simulink model "quartercar_RL_6_no_G"  (R2023a)
settings: Solver=VariableStepAuto  StartTime=0  StopTime=10  FixedStep=0.05  RelTol=1e-5  EnableMultiTasking=on
model workspace (MAT data in the model file):
  cs = 2126
  ks = 24000
  kt = 243000
  ms = 365
  mu = 43
undefined symbols (not defined in the file or in its folder): magnitude
libraries: simulink x3, slpidlib x1, rllib x1
settings Model: Creator=Administrator  LastModifiedBy=Yuk
settings SolverCC: AllowMultiTaskInputOutput=on  InsertRTBMode=Never (minimum delay)
settings DataIOCC: SaveFormat=Array
settings OptimizationCC: LifeSpan=inf
settings DebuggingCC: AlgebraicLoopMsg=none  UnderspecifiedInitializationDetection=Classic  MergeDetectMultiDrivingBlocksExec=none  SolverPrmCheckMsg=warning  UnconnectedInputMsg=warning  UnconnectedOutputMsg=warning  UnconnectedLineMsg=warning  StateNameClashWarn=warning  SFUnexpectedBacktrackingDiag=warning  SFNoUnconditionalDefaultTransitionDiag=warning  SFExecutionAtInitializationDiag=none  ArithmeticOperatorsInVariantConditions=warning
settings HardwareCC: ProdBitPerPointer=32  ProdBitPerSizeT=32  ProdBitPerPtrDiffT=32  ProdLargestAtomicFloat=None  ProdIntDivRoundTo=Undefined  ProdEndianess=Unspecified  ProdWordSize=32  ProdHWDeviceType=32-bit Generic
settings ModelReferenceCC: PropagateSignalLabelsOutOfModel=off
settings SFSimCC: SimUseLocalCustomCode=off  CustomCodeUndefinedFunction=UseInterfaceOnly  SimTargetLang=C++
settings RTWCC: RTWUseLocalCustomCode=off
settings CodeAppCC: StateflowObjectComments=on
settings GRTTargetCC: TargetLangStandard=C89/C90 (ANSI)
settings ConfigComp: CovMetricSettings=dw  CovSaveCumulativeToWorkspaceVar=on  CovSaveSingleToWorkspaceVar=on  CovExternalEMLEnable=off

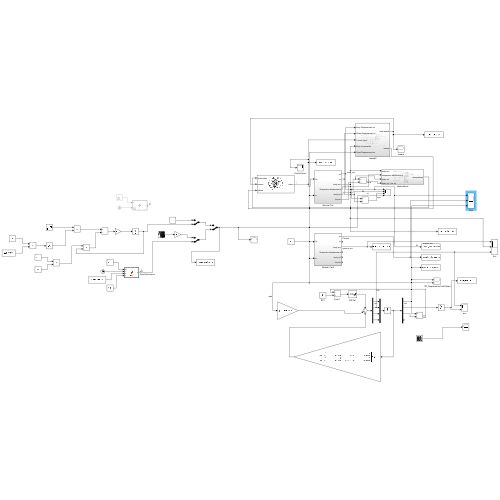
[thumbnail: Simulink's stored preview of the top-level diagram]
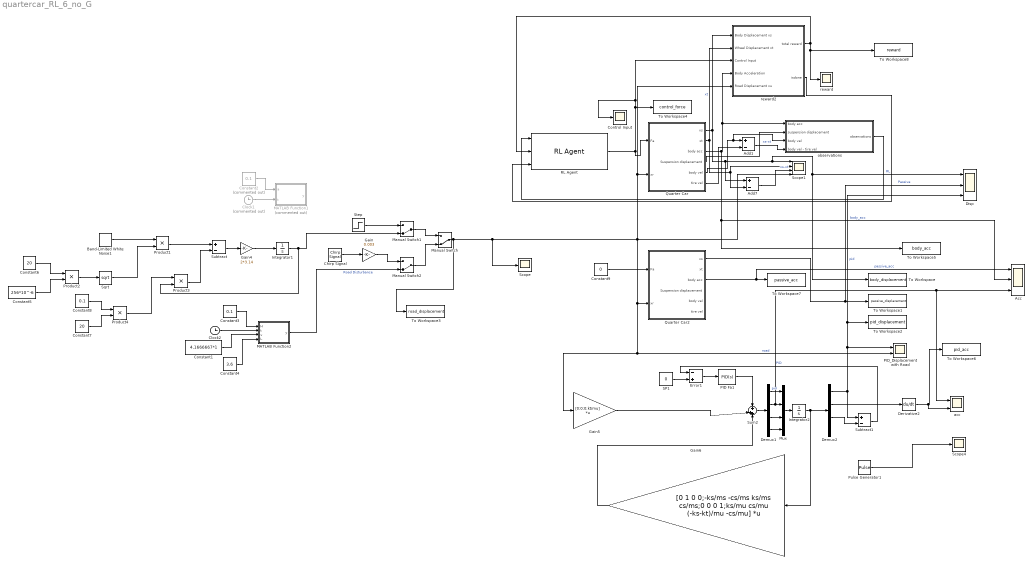
== system quartercar_RL_6_no_G ==
  Acc : Scope  NumInputPorts=3
  Add1 : Sum  Inputs=+-
  Add7 : Sum  Inputs=+-
  Band-Limited White Noise1 : simulink/Sources/Band-Limited White Noise  Cov=[5.4*10^-3]  Ts=0.1  seed=[23341]
  Chirp Signal : simulink/Sources/Chirp Signal  f1=1  T=10  f2=1
  Clock1 : Clock  Commented=on
  Clock2 : Clock
  Constant1 : Constant  Value=4.1666667*1
  Constant2 : Constant  Commented=on  Value=0.1
  Constant3 : Constant  Value=0.1
  Constant4 : Constant  Value=3.6
  Constant5 : Constant  Value=256*10^-6
  Constant6 : Constant  Value=20
  Constant7 : Constant  Value=20
  Constant8 : Constant  Value=0.1
  Constant9 : Constant  Value=0
  Control Input : Scope
  Demux1 : Demux
  Demux2 : Demux
  Derivative2 : Derivative
  Disp : Scope  NumInputPorts=3
  Error1 : Sum  Inputs=-+
  Gain : Gain  Gain=0.003
  Gain4 : Gain  Gain=2*3.14
  Gain5 : Gain  Gain=[0;0;0;kt/mu]  Multiplication=Matrix(K*u)
  Gain6 : Gain  Gain=[0 1 0 0;-ks/ms -cs/ms ks/ms cs/ms;0 0 0 1;ks/mu cs/mu (-ks-kt)/mu -cs/mu]  Multiplication=Matrix(K*u)
  Integrator1 : Integrator
  Integrator2 : Integrator
  MATLAB Function1 : MATLAB Function  Commented=on  TreatAsAtomicUnit=on
  MATLAB Function2 : MATLAB Function  TreatAsAtomicUnit=on
  Manual Switch : ManualSwitch  CurrentSetting=0
  Manual Switch1 : ManualSwitch  CurrentSetting=0
  Manual Switch2 : ManualSwitch  CurrentSetting=0
  Mux : Mux
  PID Fa1 : slpidlib/PID Controller  Controller=PID  Form=Parallel  TimeDomain=Continuous-time  UseExternalTs=off  SampleTime=1  IntegratorMethod=Forward Euler  FilterMethod=Forward Euler  ControllerParametersSource=internal  P=0.8  I=0.1  UseKiTs=off  D=0.5  N=100  UseFilter=on  TunerSelectOption=Transfer Function Based (PID Tuner App)  InitialConditionSource=internal  InitialConditionForIntegrator=0  InitialConditionForFilter=0  DifferentiatorICPrevScaledInput=0  ExternalReset=none  TrackingMode=off  Kt=1  LimitOutput=on  SatLimitsSource=internal  UpperSaturationLimit=4000  LowerSaturationLimit=-4000  LinearizeAsGain=off  AntiWindupMode=none  Kb=1  LimitIntegrator=off  UpperIntegratorSaturationLimit=inf  LowerIntegratorSaturationLimit=-inf  POutMin=[]  POutMax=[]  IOutMin=[]  IOutMax=[]  DOutMin=[]  DOutMax=[]  NOutMin=[]  NOutMax=[]  SumOutMin=[]  SumOutMax=[]  SaturationOutMin=[]  SaturationOutMax=[]  PParamMin=[]  PParamMax=[]  IParamMin=[]  IParamMax=[]  DParamMin=[]  DParamMax=[]  NParamMin=[]  NParamMax=[]  KbParamMin=[]  KbParamMax=[]  KtParamMin=[]  KtParamMax=[]  KbOutMin=[]  KbOutMax=[]  KtOutMin=[]  KtOutMax=[]  IntegratorOutMin=[]  IntegratorOutMax=[]  FilterOutMin=[]  FilterOutMax=[]  SumI1OutMin=[]  SumI1OutMax=[]  SumI2OutMin=[]  SumI2OutMax=[]  SumI3OutMin=[]  SumI3OutMax=[]  SumI4OutMin=[]  SumI4OutMax=[]  SumDOutMin=[]  SumDOutMax=[]  DifferentiatorOutMin=[]  DifferentiatorOutMax=[]  FilterDiffOutCoefMin=[]  FilterDiffOutCoefMax=[]  ReciprocalOutMin=[]  ReciprocalOutMax=[]  SumDenOutMin=[]  SumDenOutMax=[]  SumNumOutMin=[]  SumNumOutMax=[]  DivideOutMin=[]  DivideOutMax=[]  UdiffTsProdOutMin=[]  UdiffTsProdOutMax=[]  NTsProdOutMin=[]  NTsProdOutMax=[]  UintegralTsProdOutMin=[]  UintegralTsProdOutMax=[]  UngainTsProdOutMin=[]  UngainTsProdOutMax=[]  ClampingZeroOutDataTypeStr=Inherit: Inherit via back propagation  ClampingZeroOutMin=[]  ClampingZeroOutMax=[]  FilterDenConstantOutDataTypeStr=Inherit: Inherit via back propagation  FilterDenConstantOutMin=[]  FilterDenConstantOutMax=[]  PCopyOutDataTypeStr=Inherit: Inherit via back propagation  PCopyOutMin=[]  PCopyOutMax=[]  NCopyOutDataTypeStr=Inherit: Inherit via back propagation  NCopyOutMin=[]  NCopyOutMax=[]  IntegratorContinuousStateAttributes=''  IntegratorStateMustResolveToSignalObject=off  IntegratorRTWStateStorageClass=Auto  FilterContinuousStateAttributes=''  FilterStateMustResolveToSignalObject=off  FilterRTWStateStorageClass=Auto  ParallelPVariant=InternalParameters  IdealPVariant=Disabled  IVariant=InternalParameters  DVariant=InternalParameters  IntegratorVariant=Continuous  SatVariant=Enabled  AWVariant=Passthrough  PCopyVariant=Disabled  TRVariant=Disabled  FdbkBlocksVariant=Forward  IdealPFdbkVariant=Disabled  SatFdbkVariant=Disabled  DerivativeFilterVariant=ContFilter  NVariant=InternalParameters  NCopyVariant=Disabled  FilterICVariant=InternalICsFilter  IntegratorICVariant=InternalICs  ExternalResetVariant=Disabled  TRSumVariant=Passthrough  SumFdbkVariant=Disabled  SumVariant=Sum_PID  TsampFilterVariant=InternalTs  TsampNgainVariant=Passthrough  TsampIntegralVariant=Disabled_SignalSpec  ExternalSaturationOutDataTypeStr=Inherit: Same as second input
  PID_Displacement with Road : Scope  NumInputPorts=2
  Product{1..4} (4 alike) : Product
  Pulse Generator1 : DiscretePulseGenerator  PulseType=Time based  Period=10  PulseWidth=5
  Quarter Car : Subsystem
  Quarter Car2 : Subsystem
  RL Agent : rllib/RL Agent  Agent=saved_agent  ExternalActionAsInput=off  ProvideLastAction=off  ProvideCumRwd=off  TreatAsDirectFeedthrough=on  UseStrictObservationDataTypes=off
  SP1 : Constant  Value=0
  Scope : Scope
  Scope1 : Scope  NumInputPorts=4
  Scope4 : Scope
  Sqrt : Sqrt
  Step : Step  SampleTime=0
  Subtract : Sum  Inputs=+-
  Subtract1 : Sum  Inputs=+-
  Sum2 : Sum  Inputs=+|++
  To Workspace : ToWorkspace  VariableName=body_displacement  SaveFormat=Timeseries  SampleTime=-1
  To Workspace1 : ToWorkspace  VariableName=passive_displacement  SaveFormat=Timeseries  SampleTime=-1
  To Workspace2 : ToWorkspace  VariableName=pid_displacement  SaveFormat=Timeseries  SampleTime=-1
  To Workspace3 : ToWorkspace  VariableName=road_displacement  SaveFormat=Timeseries  SampleTime=-1
  To Workspace4 : ToWorkspace  VariableName=control_force  SaveFormat=Timeseries  SampleTime=-1
  To Workspace5 : ToWorkspace  VariableName=body_acc  SaveFormat=Timeseries  SampleTime=-1
  To Workspace6 : ToWorkspace  VariableName=pid_acc  SaveFormat=Timeseries  SampleTime=0.05
  To Workspace7 : ToWorkspace  VariableName=passive_acc  SaveFormat=Timeseries  SampleTime=-1
  To Workspace8 : ToWorkspace  VariableName=reward  SaveFormat=Timeseries  SampleTime=-1
  acc : Scope  NumInputPorts=2
  observations : Subsystem
  reward : Scope
  reward2 : Subsystem
  wires:
  Quarter Car/1(xs) -> reward2/1(Body Displacement xs), Add7/1, To Workspace/1, Disp/1, Scope1/1  "RL"
  Quarter Car/2(xt) -> Add7/2, Scope1/2, reward2/2(Wheel Displacement xt)  "xt"
  Add7/1 -> Scope1/3  "xs-xt"
  Constant2/1 -> MATLAB Function1/1(a)
  Clock1/1 -> MATLAB Function1/2(t)
  reward2/1(total reward) -> reward/1, To Workspace8/1, RL Agent/2
  Quarter Car/3(body acc) -> To Workspace5/1, Acc/2, reward2/4(Body Acceleration), observations/1(body acc)  "body_acc"
  observations/1(observations) -> RL Agent/1
  reward2/2(isdone) -> RL Agent/3
  Quarter Car/4(Suspension displacement) -> observations/2(suspension displacement)
  Quarter Car/5(body vel) -> observations/3(body vel), Add1/1
  Quarter Car/6(tire vel) -> Add1/2
  Add1/1 -> observations/4(body vel - tire vel)  "xs-xt"
  RL Agent/1 -> Quarter Car/1(Fa), To Workspace4/1, Control Input/1, reward2/3(Control Input)
  Quarter Car2/1(xs) -> Disp/2, To Workspace1/1  "Passive"
  Quarter Car2/3(body acc) -> Acc/1, To Workspace7/1  "passive_acc"
  Manual Switch1/1 -> Manual Switch/1
  Integrator1/1 -> Product3/2, Manual Switch1/2
  Constant5/1 -> Product2/2
  Sqrt/1 -> Product1/2
  Constant6/1 -> Product2/1
  Product2/1 -> Sqrt/1
  Constant7/1 -> Product4/2
  Gain4/1 -> Integrator1/1
  Product1/1 -> Subtract/1
  Band-Limited White Noise1/1 -> Product1/1
  Product3/1 -> Subtract/2
  Subtract/1 -> Gain4/1
  MATLAB Function2/1(y) -> Manual Switch2/2  "Road Disturbance"
  Constant1/1 -> MATLAB Function2/3(v)
  Clock2/1 -> MATLAB Function2/2(t)
  Constant3/1 -> MATLAB Function2/1(H)
  Constant4/1 -> MATLAB Function2/4(L)
  Manual Switch2/1 -> Manual Switch/2
  Constant8/1 -> Product4/1
  Product4/1 -> Product3/1
  Constant9/1 -> Quarter Car2/1(Fa)
  Step/1 -> Manual Switch1/1
  Gain6/1 -> Sum2/3
  Subtract1/1 -> Error1/1  "PID"
  Sum2/1 -> Demux1/1
  Demux2/1 -> PID_Displacement with Road/1, Disp/3, To Workspace2/1, Subtract1/1  "pid"
  Demux2/3 -> Subtract1/2
  Gain5/1 -> Sum2/2
  Manual Switch/1 -> Scope/1, Gain5/1, PID_Displacement with Road/2, Quarter Car2/2(xr), Scope1/4, reward2/5(Road Displacement xu), Quarter Car/2(xr), To Workspace3/1  "road"
  SP1/1 -> Error1/2
  PID Fa1/1 -> Sum2/1
  Error1/1 -> PID Fa1/1
  Integrator2/1 -> Gain6/1, Demux2/1
  Demux2/2 -> Derivative2/1
  Derivative2/1 -> acc/2, To Workspace6/1
  Gain/1 -> Manual Switch2/1
  Chirp Signal/1 -> Gain/1
  Demux1/1 -> Mux/1  "pid"
  Demux1/2 -> acc/1, Acc/3, Mux/2
  Demux1/3 -> Mux/3
  Demux1/4 -> Mux/4
  Mux/1 -> Integrator2/1
  Pulse Generator1/1 -> Scope4/1

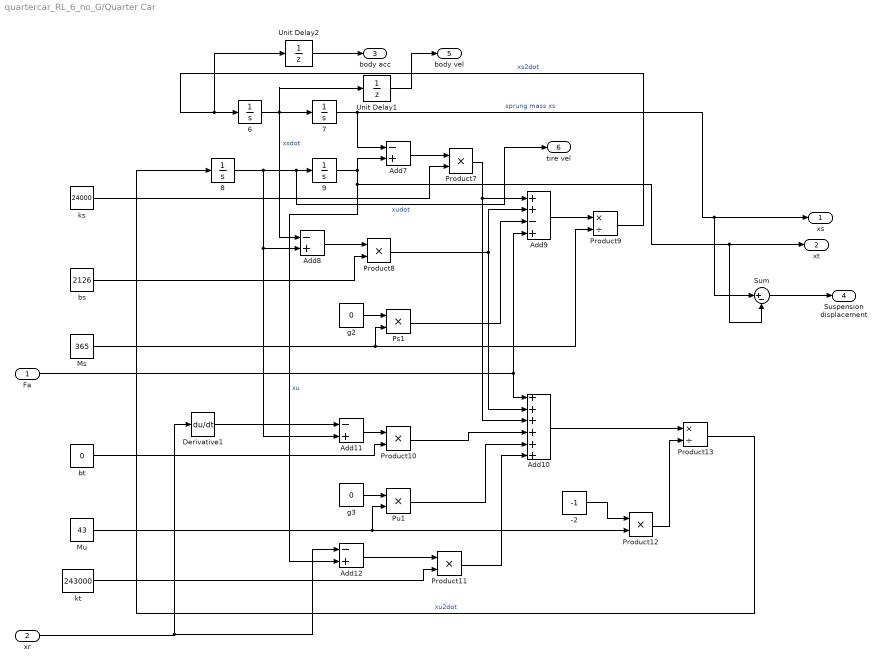
== system quartercar_RL_6_no_G/Quarter Car ==
  Fa : Inport
  xr : Inport  Port=2
  -2 : Constant  Value=-1
  {6..9} (4 alike) : Integrator
  Add10 : Sum  Inputs=++++++
  Add{7..8,11..12} (4 alike) : Sum  Inputs=-+
  Add9 : Sum  Inputs=++-+
  Derivative1 : Derivative
  Ms : Constant  Value=365
  Mu : Constant  Value=43
  Product{7..8,10..12} (5 alike) : Product
  Product13 : Product  Inputs=*/
  Product9 : Product  Inputs=*/
  Ps1 : Product
  Pu1 : Product
  Sum : Sum  Inputs=|+-
  Unit Delay1 : UnitDelay  SampleTime=-1  HasFrameUpgradeWarning=on
  Unit Delay2 : UnitDelay  SampleTime=-1  HasFrameUpgradeWarning=on
  bs : Constant  Value=2126
  bt : Constant  Value=0
  g2 : Constant  Value=0
  g3 : Constant  Value=0
  ks : Constant  Value=24000
  kt : Constant  Value=243000
  xs : Outport
  xt : Outport  Port=2
  body acc : Outport  Port=3
  Suspension displacement : Outport  Port=4
  body vel : Outport  Port=5
  tire vel : Outport  Port=6
  wires:
  g2/1 -> Ps1/1
  Product12/1 -> Product13/2
  g3/1 -> Pu1/1
  Ps1/1 -> Add9/3
  Add10/1 -> Product13/1
  -2/1 -> Product12/1
  Mu/1 -> Pu1/2, Product12/2
  Product11/1 -> Add10/6
  Add12/1 -> Product11/1
  kt/1 -> Product11/2
  xr/1 -> Add12/1, Derivative1/1
  Pu1/1 -> Add10/5
  Product10/1 -> Add10/4
  Add11/1 -> Product10/1
  bt/1 -> Product10/2
  Derivative1/1 -> Add11/1
  Ms/1 -> Product9/2, Ps1/2
  Add9/1 -> Product9/1
  Fa/1 -> Add10/1, Add9/4
  Product8/1 -> Add10/2, Add9/2
  Product7/1 -> Add10/3, Add9/1
  bs/1 -> Product8/2
  Add8/1 -> Product8/1
  ks/1 -> Product7/2
  Add7/1 -> Product7/1
  9/1 -> Add12/2, Sum/2, xt/1, Add7/2  "xu"
  Product13/1 -> 8/1  "xu2dot"
  8/1 -> tire vel/1, 9/1, Add8/2, Add11/2  "xudot"
  7/1 -> Add7/1, Sum/1, xs/1  "sprung mass xs"
  Product9/1 -> Unit Delay2/1, 6/1  "xs2dot"
  6/1 -> Unit Delay1/1, 7/1, Add8/1  "xsdot"
  Sum/1 -> Suspension displacement/1
  Unit Delay1/1 -> body vel/1
  Unit Delay2/1 -> body acc/1

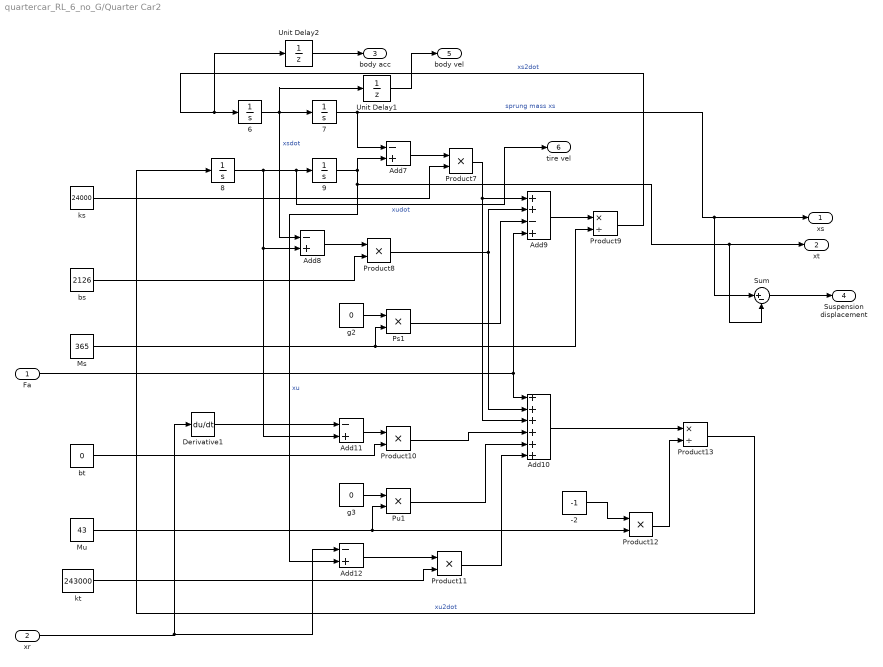
== system quartercar_RL_6_no_G/Quarter Car2 ==
  Fa : Inport
  xr : Inport  Port=2
  -2 : Constant  Value=-1
  {6..9} (4 alike) : Integrator
  Add10 : Sum  Inputs=++++++
  Add{7..8,11..12} (4 alike) : Sum  Inputs=-+
  Add9 : Sum  Inputs=++-+
  Derivative1 : Derivative
  Ms : Constant  Value=365
  Mu : Constant  Value=43
  Product{7..8,10..12} (5 alike) : Product
  Product13 : Product  Inputs=*/
  Product9 : Product  Inputs=*/
  Ps1 : Product
  Pu1 : Product
  Sum : Sum  Inputs=|+-
  Unit Delay1 : UnitDelay  SampleTime=-1  HasFrameUpgradeWarning=on
  Unit Delay2 : UnitDelay  SampleTime=-1  HasFrameUpgradeWarning=on
  bs : Constant  Value=2126
  bt : Constant  Value=0
  g2 : Constant  Value=0
  g3 : Constant  Value=0
  ks : Constant  Value=24000
  kt : Constant  Value=243000
  xs : Outport
  xt : Outport  Port=2
  body acc : Outport  Port=3
  Suspension displacement : Outport  Port=4
  body vel : Outport  Port=5
  tire vel : Outport  Port=6
  wires:
  g2/1 -> Ps1/1
  Product12/1 -> Product13/2
  g3/1 -> Pu1/1
  Ps1/1 -> Add9/3
  Add10/1 -> Product13/1
  -2/1 -> Product12/1
  Mu/1 -> Pu1/2, Product12/2
  Product11/1 -> Add10/6
  Add12/1 -> Product11/1
  kt/1 -> Product11/2
  xr/1 -> Add12/1, Derivative1/1
  Pu1/1 -> Add10/5
  Product10/1 -> Add10/4
  Add11/1 -> Product10/1
  bt/1 -> Product10/2
  Derivative1/1 -> Add11/1
  Ms/1 -> Product9/2, Ps1/2
  Add9/1 -> Product9/1
  Fa/1 -> Add10/1, Add9/4
  Product8/1 -> Add10/2, Add9/2
  Product7/1 -> Add10/3, Add9/1
  bs/1 -> Product8/2
  Add8/1 -> Product8/1
  ks/1 -> Product7/2
  Add7/1 -> Product7/1
  9/1 -> Add12/2, Sum/2, xt/1, Add7/2  "xu"
  Product13/1 -> 8/1  "xu2dot"
  8/1 -> tire vel/1, 9/1, Add8/2, Add11/2  "xudot"
  7/1 -> Add7/1, Sum/1, xs/1  "sprung mass xs"
  Product9/1 -> Unit Delay2/1, 6/1  "xs2dot"
  6/1 -> Unit Delay1/1, 7/1, Add8/1  "xsdot"
  Sum/1 -> Suspension displacement/1
  Unit Delay1/1 -> body vel/1
  Unit Delay2/1 -> body acc/1

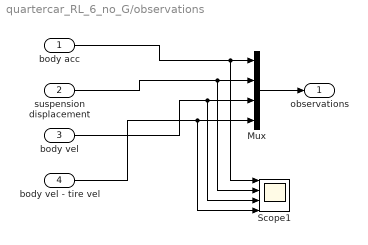
== system quartercar_RL_6_no_G/observations ==
  body acc : Inport
  suspension displacement : Inport  Port=2
  body vel : Inport  Port=3
  body vel - tire vel : Inport  Port=4
  Mux : Mux
  Scope1 : Scope  NumInputPorts=4
  observations : Outport
  wires:
  body acc/1 -> Scope1/1, Mux/1
  Mux/1 -> observations/1
  body vel/1 -> Scope1/3, Mux/3
  suspension displacement/1 -> Scope1/2, Mux/2
  body vel - tire vel/1 -> Scope1/4, Mux/4

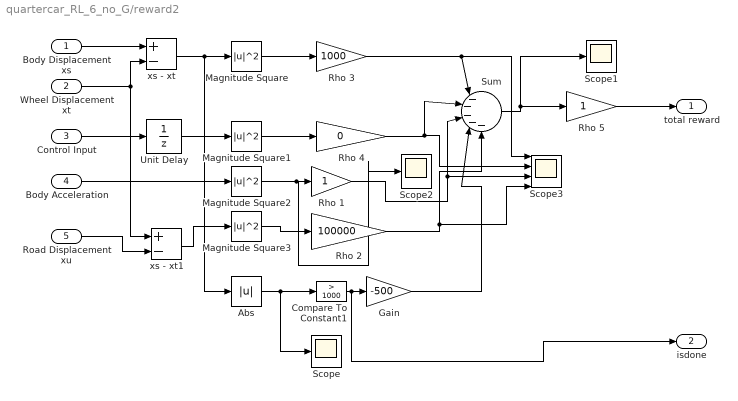
== system quartercar_RL_6_no_G/reward2 ==
  Body Displacement xs : Inport
  Wheel Displacement xt : Inport  Port=2
  Control Input : Inport  Port=3
  Body Acceleration : Inport  Port=4
  Road Displacement xu : Inport  Port=5
  Abs : Abs  SaturateOnIntegerOverflow=off
  Compare To Constant1 : simulink/Logic and Bit Operations/Compare To Constant  relop=>  const=1000  OutDataTypeStr=boolean
  Gain : Gain  Gain=-500
  Magnitude Square{,1..3} (4 alike) : Math  Operator=magnitude^2  SignedPower=on  RndMeth=Zero
  Rho 1 : Gain
  Rho 2 : Gain  Gain=100000
  Rho 3 : Gain  Gain=1000
  Rho 4 : Gain  Gain=0
  Rho 5 : Gain
  Scope : Scope
  Scope1 : Scope
  Scope2 : Scope
  Scope3 : Scope  NumInputPorts=4
  Sum : Sum  Inputs=|-----
  Unit Delay : UnitDelay  SampleTime=-1  HasFrameUpgradeWarning=on
  xs - xt : Sum  Inputs=+-
  xs - xt1 : Sum  Inputs=+-
  total reward : Outport
  isdone : Outport  Port=2
  wires:
  Wheel Displacement xt/1 -> xs - xt1/1, xs - xt/2
  Body Displacement xs/1 -> xs - xt/1
  Magnitude Square2/1 -> Scope2/1, Rho 1/1
  xs - xt/1 -> Magnitude Square/1, Abs/1
  Magnitude Square/1 -> Rho 3/1
  Control Input/1 -> Unit Delay/1
  Unit Delay/1 -> Magnitude Square1/1
  Rho 3/1 -> Scope3/1, Sum/1
  Sum/1 -> Rho 5/1, Scope1/1
  Compare To Constant1/1 -> isdone/1, Gain/1
  Rho 1/1 -> Scope3/3, Sum/3
  Gain/1 -> Sum/4
  Body Acceleration/1 -> Magnitude Square2/1
  Rho 5/1 -> total reward/1
  Abs/1 -> Scope/1, Compare To Constant1/1
  Rho 4/1 -> Scope3/2, Sum/2
  Magnitude Square1/1 -> Rho 4/1
  Road Displacement xu/1 -> xs - xt1/2
  xs - xt1/1 -> Magnitude Square3/1
  Magnitude Square3/1 -> Rho 2/1
  Rho 2/1 -> Scope3/4, Sum/5

== matlab function quartercar_RL_6_no_G/MATLAB Function2 ==
  data: H input; y output; t input; v input; L input
function y = fcn(H,t,v,L)
% CODE GENERATION
if (0.5<t) && (t<L/v+0.5)
    
  y=H/2*(1-cos((2*pi*v/L)*(t-0.5)));
% w = 2*pi*v/L;
%   y=H*(1-cos(w*t));

else
    y=0;
end
out=y;

== matlab function quartercar_RL_6_no_G/MATLAB Function1 ==
  data: a input; y output; t input
function y = fcn(a,t)
% CODE GENERATION
if (t>=0.5 && t<=1.5)
    
    % y= a*(1-cos(2*pi*t))/2;
    y= a/2*(1+cos(2*pi*t));
    % y= a-(a/2*(1-cos(2*pi*t)));
% elseif (t>=5.5 && t<=6.5)
%     y= 0.07/2*(1+cos(2*pi*t));

else
    y=0;
end
out=y;
